simulink model "BMS_SIL_Protection_Test"  (R2025b)
settings: Solver=FixedStepDiscrete  StartTime=0.0  StopTime=6  FixedStep=Ts  RelTol=1e-3
undefined symbols (not defined in the file): Ts
settings Model: Creator=Khadija  LastModifiedBy=Khadija

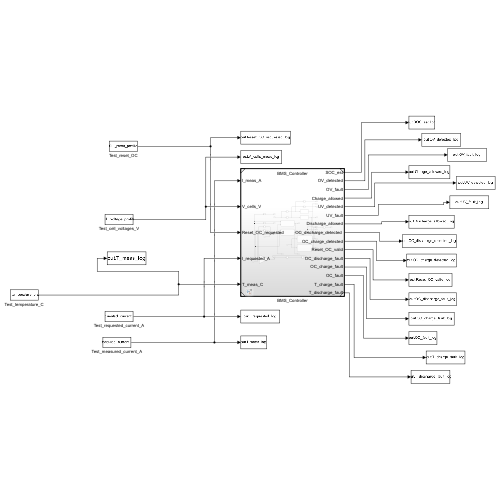
[thumbnail: Simulink's stored preview of the top-level diagram]
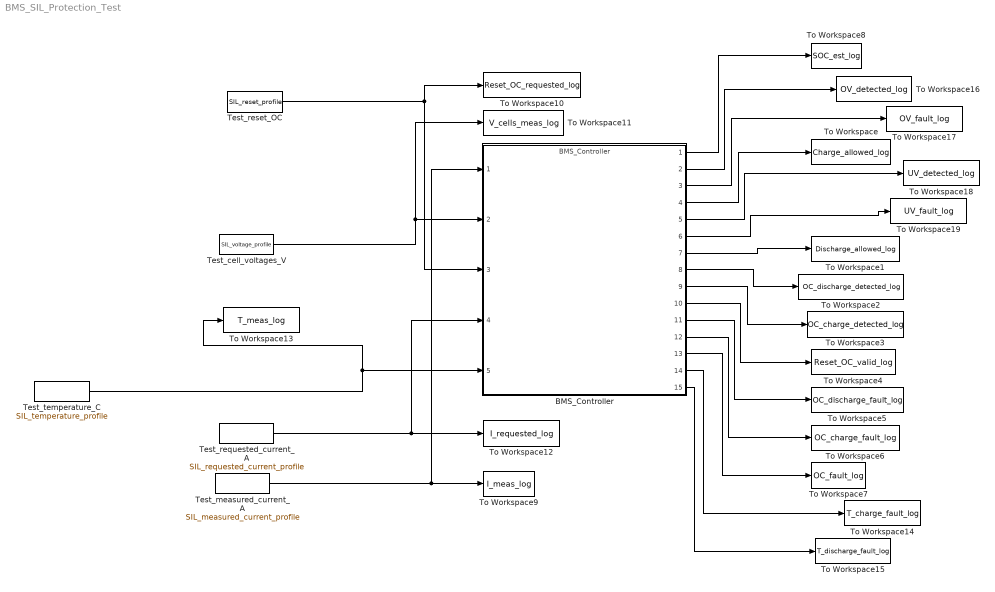
== system BMS_SIL_Protection_Test ==
  BMS_Controller : ModelReference  ModelNameDialog=BMS_Controller.slx  SimulationMode=Normal  ModelReferenceVersion=1.41
  Test_cell_voltages_V : FromWorkspace  VariableName=SIL_voltage_profile  OutDataTypeStr=double  SampleTime=Ts  Interpolate=off  OutputAfterFinalValue=Holding final value
  Test_measured_current_A : FromWorkspace  VariableName=SIL_measured_current_profile  OutDataTypeStr=double  SampleTime=Ts  Interpolate=off  OutputAfterFinalValue=Holding final value
  Test_requested_current_A : FromWorkspace  VariableName=SIL_requested_current_profile  OutDataTypeStr=double  SampleTime=Ts  Interpolate=off  OutputAfterFinalValue=Holding final value
  Test_reset_OC : FromWorkspace  VariableName=SIL_reset_profile  SampleTime=Ts  Interpolate=off  OutputAfterFinalValue=Holding final value
  Test_temperature_C : FromWorkspace  VariableName=SIL_temperature_profile  OutDataTypeStr=double  SampleTime=Ts  Interpolate=off  OutputAfterFinalValue=Holding final value
  To Workspace : ToWorkspace  VariableName=Charge_allowed_log  SaveFormat=Timeseries  SampleTime=-1
  To Workspace1 : ToWorkspace  VariableName=Discharge_allowed_log  SaveFormat=Timeseries  SampleTime=-1
  To Workspace10 : ToWorkspace  VariableName=Reset_OC_requested_log  SaveFormat=Timeseries  SampleTime=-1
  To Workspace11 : ToWorkspace  VariableName=V_cells_meas_log  SaveFormat=Timeseries  SampleTime=-1
  To Workspace12 : ToWorkspace  VariableName=I_requested_log  SaveFormat=Timeseries  SampleTime=-1
  To Workspace13 : ToWorkspace  VariableName=T_meas_log  SaveFormat=Timeseries  SampleTime=-1
  To Workspace14 : ToWorkspace  VariableName=T_charge_fault_log  SaveFormat=Timeseries  SampleTime=-1
  To Workspace15 : ToWorkspace  VariableName=T_discharge_fault_log  SaveFormat=Timeseries  SampleTime=-1
  To Workspace16 : ToWorkspace  VariableName=OV_detected_log  SaveFormat=Timeseries  SampleTime=-1
  To Workspace17 : ToWorkspace  VariableName=OV_fault_log  SaveFormat=Timeseries  SampleTime=-1
  To Workspace18 : ToWorkspace  VariableName=UV_detected_log  SaveFormat=Timeseries  SampleTime=-1
  To Workspace19 : ToWorkspace  VariableName=UV_fault_log  SaveFormat=Timeseries  SampleTime=-1
  To Workspace2 : ToWorkspace  VariableName=OC_discharge_detected_log  SaveFormat=Timeseries  SampleTime=-1
  To Workspace3 : ToWorkspace  VariableName=OC_charge_detected_log  SaveFormat=Timeseries  SampleTime=-1
  To Workspace4 : ToWorkspace  VariableName=Reset_OC_valid_log  SaveFormat=Timeseries  SampleTime=-1
  To Workspace5 : ToWorkspace  VariableName=OC_discharge_fault_log  SaveFormat=Timeseries  SampleTime=-1
  To Workspace6 : ToWorkspace  VariableName=OC_charge_fault_log  SaveFormat=Timeseries  SampleTime=-1
  To Workspace7 : ToWorkspace  VariableName=OC_fault_log  SaveFormat=Timeseries  SampleTime=-1
  To Workspace8 : ToWorkspace  VariableName=SOC_est_log  SaveFormat=Timeseries  SampleTime=-1
  To Workspace9 : ToWorkspace  VariableName=I_meas_log  SaveFormat=Timeseries  SampleTime=-1
  wires:
  Test_reset_OC/1 -> To Workspace10/1, BMS_Controller/3
  Test_requested_current_A/1 -> To Workspace12/1, BMS_Controller/4
  Test_cell_voltages_V/1 -> To Workspace11/1, BMS_Controller/2
  Test_measured_current_A/1 -> BMS_Controller/1, To Workspace9/1
  BMS_Controller/1 -> To Workspace8/1
  BMS_Controller/2 -> To Workspace16/1
  BMS_Controller/3 -> To Workspace17/1
  BMS_Controller/7 -> To Workspace1/1
  BMS_Controller/6 -> To Workspace19/1
  BMS_Controller/5 -> To Workspace18/1
  BMS_Controller/4 -> To Workspace/1
  BMS_Controller/11 -> To Workspace5/1
  BMS_Controller/10 -> To Workspace4/1
  BMS_Controller/9 -> To Workspace3/1
  BMS_Controller/8 -> To Workspace2/1
  BMS_Controller/13 -> To Workspace7/1
  BMS_Controller/12 -> To Workspace6/1
  Test_temperature_C/1 -> To Workspace13/1, BMS_Controller/5
  BMS_Controller/14 -> To Workspace14/1
  BMS_Controller/15 -> To Workspace15/1
